simulink model "DK_V3_Steuerung_ohne_Regler"  (R2025b)
settings: Solver=ode23tb  StartTime=0.0  StopTime=2.0  MaxStep=1e-3  RelTol=1e-4  AbsTol=1e-6
settings Model: Creator=johan  LastModifiedBy=johan

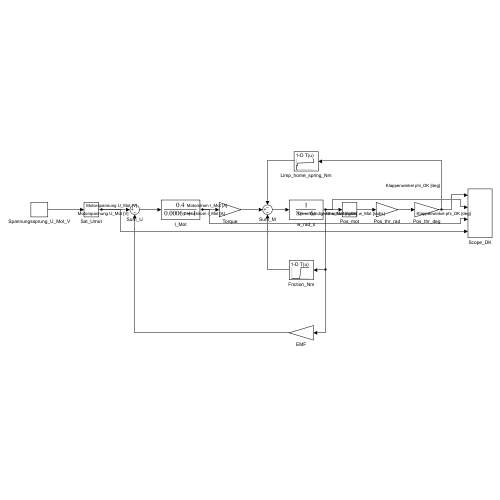
[thumbnail: Simulink's stored preview of the top-level diagram]
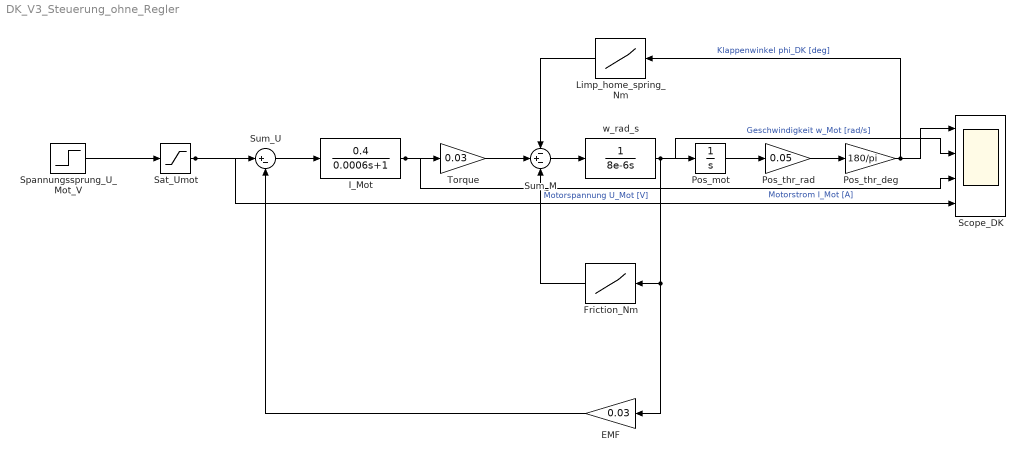
== system DK_V3_Steuerung_ohne_Regler ==
  EMF : Gain  Gain=0.03
  Friction_Nm : Lookup_n-D  NumberOfTableDimensions=1  BreakpointsForDimension1=[-10, -1, 1, 10]  Table=[-0.01, -0.01, 0.01, 0.01]  InternalRulePriority=Speed  RndMeth=Simplest
  I_Mot : TransferFcn  Numerator=[0.4]  Denominator=[0.0006 1]
  Limp_home_spring_Nm : Lookup_n-D  NumberOfTableDimensions=1  BreakpointsForDimension1=[-0.1, 0, 4.9, 5.1, 90, 90.1]  Table=[-0.1, -0.0253, -0.025, 0.025, 0.029, 0.1]  InternalRulePriority=Speed  RndMeth=Simplest
  Pos_mot : Integrator  InitialCondition=5 * (pi/180) / 0.05
  Pos_thr_deg : Gain  Gain=180/pi
  Pos_thr_rad : Gain  Gain=0.05
  Sat_Umot : Saturate  UpperLimit=12  LowerLimit=-12
  Scope_DK : Scope  NumInputPorts=4
  Spannungssprung_U_Mot_V : Step  Time=0.1  After=6  SampleTime=0
  Sum_M : Sum  Inputs=-+-
  Sum_U : Sum  Inputs=|+-
  Torque : Gain  Gain=0.03
  w_rad_s : TransferFcn  Denominator=[8e-6 0]
  wires:
  Spannungssprung_U_Mot_V/1 -> Sat_Umot/1
  Sat_Umot/1 -> Sum_U/1, Scope_DK/4  "Motorspannung U_Mot [V]"
  Sum_U/1 -> I_Mot/1
  I_Mot/1 -> Torque/1, Scope_DK/3  "Motorstrom I_Mot [A]"
  Torque/1 -> Sum_M/2
  Sum_M/1 -> w_rad_s/1
  w_rad_s/1 -> Friction_Nm/1, EMF/1, Pos_mot/1, Scope_DK/2  "Geschwindigkeit w_Mot [rad/s]"
  Pos_mot/1 -> Pos_thr_rad/1
  Pos_thr_rad/1 -> Pos_thr_deg/1
  Pos_thr_deg/1 -> Limp_home_spring_Nm/1, Scope_DK/1  "Klappenwinkel phi_DK [deg]"
  Limp_home_spring_Nm/1 -> Sum_M/1
  Friction_Nm/1 -> Sum_M/3
  EMF/1 -> Sum_U/2
